simulink model "Controller_damping_cbf_22Franka"  (R2022b)
settings: Solver=FixedStepDiscrete  StartTime=0.0  StopTime=inf  FixedStep=0.001  RelTol=1e-3
PreLoadFcn:
  | set_param(gcs, 'RTWSystemTargetFile', 'franka_emika_panda.tlc');
  | 
  | demos_common_configs();
  | collision_behavior = ones(1,52)*100;
values from neighbouring files (symbols this model uses):
  b_sg = fliplr(B(end, :))    [init_damping_cbf.m]
  cbf_damping_params = [cbf_p_ths; cbf_v_ths; cbf_v_0; cbf_gamma; cbf_d_max;                        cbf_w_lin; cbf_w_quad; plane_normal; plane_offset;                        cbf_latch_entry; cbf_zone_hyst; cbf_latch_alpha; cbf_clip_drift;                        cbf_tau_rate; cbf_dt; cbf_gamma_pos_scale]    [init_damping_cbf.m]
  cbf_kappa = 0.85 * cbf_d_max / cbf_rho_eff    (= 82.6388888889)    [init_damping_cbf.m]
  cbf_stiff_decouple = 0    [init_damping_cbf.m]
  Dn = 20 * ones(7,1)    [init_damping_cbf.m]
  H_home = getTransform(Franka_robot, q_home, 'panda_link8', 'panda_link0')    [init_damping_cbf.m]
  Kn = 0 * ones(7,1)    [init_damping_cbf.m]
  plane_normal = [0.0; 0.0; 1.0]    [init_damping_cbf.m]
  q_home = q_init    [init_damping_cbf.m]
  q_init = [0 0  0  -(2/4)*pi  0  pi/2  -pi/4]'    [init_damping_cbf.m]
undefined symbols (not defined in the file or in its folder): DiscIntNeverNeededParam, Fext_mag
libraries: matrix_library x3, franka_simulink_library x2, Robotics_lib x1
(part 3 of 8)

== matlab function Controller_damping_cbf_22Franka/task space controller/MATLAB Function2 ==
  data: H_IT input; x_c output size=1; v_c output size=1; V_tilde input; lambda_mat input; n_hp input; m_c output size=1; xTableHight input; eef_height input
function [x_c, v_c, m_c] = fcn(H_IT, V_tilde, lambda_mat, n_hp, xTableHight, eef_height)

auxMat = zeros(4,4);
auxMat(3,4) = -xTableHight;

H = H_IT*[eye(3), [0;0;eef_height];zeros(1,3),1] + auxMat;

x_c = transpose(n_hp)*[H(1:3,4);zeros(3,1)];

v_c = transpose(n_hp)*V_tilde;




lambda_inv = lambda_mat\eye(6);
lambda_inv = (lambda_inv + transpose(lambda_inv))./2;

tmp3 = transpose(n_hp)*lambda_inv*n_hp;
m_c = tmp3\eye(1);


end

== matlab function Controller_damping_cbf_22Franka/Dynamic Parameters/End Effector ==
  data: q input; H_0e output
function H_0e = H_0e(q)
% Author: TU Wien, ACIN Robotics group
% Optimized and generated from Maple
  H_0e = zeros(4,4);
  t4449 = q(6);
  t4435 = sin(t4449);
  t4442 = cos(t4449);
  t4431 = 0.107e0 * t4435 + 0.88e-1 * t4442;
  t4450 = q(5);
  t4436 = sin(t4450);
  t4452 = q(3);
  t4438 = sin(t4452);
  t4491 = t4438 * t4436;
  t4499 = t4431 * t4491;
  t4430 = 0.107e0 * t4442 - 0.88e-1 * t4435 - 0.384e0;
  t4451 = q(4);
  t4437 = sin(t4451);
  t4498 = -t4430 * t4437 - 0.825e-1;
  t4443 = cos(t4450);
  t4427 = t4431 * t4443 - 0.825e-1;
  t4444 = cos(t4451);
  t4497 = t4427 * t4444;
  t4495 = t4430 * t4444;
  t4448 = q(7);
  t4434 = sin(t4448);
  t4454 = q(1);
  t4440 = sin(t4454);
  t4494 = t4434 * t4440;
  t4493 = t4436 * t4437;
  t4492 = t4437 * t4435;
  t4490 = t4438 * t4442;
  t4489 = t4438 * t4443;
  t4441 = cos(t4448);
  t4488 = t4440 * t4441;
  t4487 = t4443 * t4437;
  t4486 = t4443 * t4444;
  t4445 = cos(t4452);
  t4485 = t4443 * t4445;
  t4484 = t4444 * t4435;
  t4483 = t4445 * t4436;
  t4482 = t4445 * t4437;
  t4481 = t4445 * t4444;
  t4453 = q(2);
  t4439 = sin(t4453);
  t4446 = cos(t4453);
  t4467 = t4436 * t4481;
  t4458 = (t4467 + t4489) * t4446;
  t4478 = t4434 * t4493;
  t4480 = t4434 * t4458 + t4439 * t4478;
  t4479 = t4431 * t4483;
  t4477 = t4442 * t4487;
  t4476 = t4436 * t4490;
  t4475 = t4444 * t4491;
  t4474 = t4441 * t4493;
  t4473 = t4437 * t4490;
  t4472 = t4442 * t4486;
  t4471 = t4442 * t4483;
  t4470 = t4440 * t4485;
  t4469 = t4438 * t4486;
  t4468 = t4443 * t4481;
  t4466 = t4427 * t4437 + 0.316e0;
  t4465 = t4497 - t4498;
  t4464 = -0.1e1 * t4497 + t4498;
  t4463 = t4477 + t4484;
  t4462 = t4472 - 0.1e1 * t4492;
  t4461 = -0.1e1 * t4472 + t4492;
  t4460 = -0.1e1 * t4477 - 0.1e1 * t4484;
  t4459 = -0.1e1 * t4467 - 0.1e1 * t4489;
  t4447 = cos(t4454);
  t4457 = (t4475 - 0.1e1 * t4485) * t4447;
  t4456 = t4438 * t4462 + t4471;
  t4455 = -0.1e1 * t4471 + t4461 * t4438;
  t4425 = t4445 * t4461 + t4476;
  t4424 = t4462 * t4445 - 0.1e1 * t4476;
  t4423 = ((-0.1e1 * t4491 + t4468) * t4446 + t4439 * t4487) * t4435 + (t4446 * t4482 - 0.1e1 * t4439 * t4444) * t4442;
  t4422 = t4424 * t4446 + t4439 * t4463;
  t4421 = (t4425 * t4446 + t4439 * t4460) * t4434 + t4441 * t4458 + t4439 * t4474;
  t4420 = (t4465 * t4445 - 0.1e1 * t4499) * t4446 + (-0.1e1 * t4495 + t4466) * t4439;
  H_0e(1,3) = t4423 * t4447 + ((-0.1e1 * t4483 - 0.1e1 * t4469) * t4435 - 0.1e1 * t4473) * t4440;
  H_0e(4,1) = 0.0e0;
  H_0e(4,3) = 0.0e0;
  H_0e(3,1) = (t4425 * t4439 + t4446 * t4463) * t4441 + t4459 * t4434 * t4439 + t4446 * t4478;
  H_0e(2,1) = (t4422 * t4440 + t4447 * t4456) * t4441 + t4480 * t4440 + t4434 * t4457;
  H_0e(4,4) = 0.1e1;
  H_0e(3,2) = (t4424 * t4434 + t4441 * t4459) * t4439 + (t4434 * t4460 + t4474) * t4446;
  H_0e(3,4) = (t4445 * t4464 + t4499) * t4439 + 0.333e0 + (t4466 - t4495) * t4446;
  H_0e(2,3) = t4423 * t4440 + ((t4469 + t4483) * t4435 + t4473) * t4447;
  H_0e(2,4) = t4420 * t4440 + (t4438 * t4465 + t4479) * t4447;
  H_0e(4,2) = 0.0e0;
  H_0e(2,2) = t4434 * t4447 * t4455 + t4421 * t4440 + t4441 * t4457;
  H_0e(1,1) = (t4422 * t4441 + t4480) * t4447 + t4455 * t4488 - 0.1e1 * t4475 * t4494 + t4434 * t4470;
  H_0e(3,3) = ((t4491 - 0.1e1 * t4468) * t4435 - 0.1e1 * t4442 * t4482) * t4439 + (-0.1e1 * t4442 * t4444 + t4435 * t4487) * t4446;
  H_0e(1,4) = t4420 * t4447 + (-0.1e1 * t4479 + t4464 * t4438) * t4440;
  H_0e(1,2) = t4421 * t4447 + t4456 * t4494 - 0.1e1 * t4475 * t4488 + t4441 * t4470;
end

== matlab function Controller_damping_cbf_22Franka/Dynamic Parameters/End Effector1 ==
  data: q_state input; H_0e output
function H_0e = Franka_EndEffectorPos(q_state)
% Author: TU Wien, ACIN Robotics group
% Optimized and generated from Maple
  H_0e = zeros(4,4);

  t30 = q_state(6);
  t16 = sin(t30);
  t23 = cos(t30);
  t12 = 0.1070e0 * t16 + 0.88e-1 * t23;
  t31 = q_state(5);
  t17 = sin(t31);
  t33 = q_state(3);
  t19 = sin(t33);
  t71 = t19 * t17;
  t80 = t12 * t71;
  t11 = 0.1070e0 * t23 - 0.88e-1 * t16 - 0.384e0;
  t32 = q_state(4);
  t18 = sin(t32);
  t79 = -t11 * t18 - 0.825e-1;
  t25 = cos(t32);
  t24 = cos(t31);
  t8 = t12 * t24 - 0.825e-1;
  t78 = t8 * t25;
  t29 = q_state(7);
  t15 = sin(t29);
  t34 = q_state(2);
  t20 = sin(t34);
  t27 = cos(t34);
  t26 = cos(t33);
  t61 = t26 * t25;
  t57 = t17 * t61;
  t69 = t19 * t24;
  t39 = (t57 + t69) * t27;
  t72 = t17 * t18;
  t60 = t15 * t72;
  t77 = t15 * t39 + t20 * t60;
  t75 = t11 * t25;
  t35 = q_state(1);
  t21 = sin(t35);
  t74 = t15 * t21;
  t73 = t18 * t16;
  t70 = t19 * t23;
  t22 = cos(t29);
  t68 = t21 * t22;
  t67 = t24 * t18;
  t66 = t24 * t26;
  t65 = t16 * t25;
  t64 = t25 * t24;
  t63 = t26 * t17;
  t62 = t26 * t18;
  t59 = t12 * t63;
  t58 = t25 * t71;
  t56 = t17 * t70;
  t55 = t22 * t72;
  t54 = t18 * t70;
  t53 = t23 * t67;
  t52 = t23 * t64;
  t51 = t23 * t63;
  t50 = t21 * t66;
  t49 = t19 * t64;
  t48 = t24 * t61;
  t47 = t8 * t18 + 0.316e0;
  t46 = t78 - t79;
  t45 = t53 + t65;
  t44 = -0.1e1 * t73 + t52;
  t43 = -0.1e1 * t52 + t73;
  t42 = -0.1e1 * t78 + t79;
  t41 = -0.1e1 * t57 - 0.1e1 * t69;
  t40 = -0.1e1 * t53 - 0.1e1 * t65;
  t28 = cos(t35);
  t38 = (t58 - 0.1e1 * t66) * t28;
  t37 = t19 * t44 + t51;
  t36 = -0.1e1 * t51 + t43 * t19;
  t6 = t26 * t43 + t56;
  t5 = t44 * t26 - 0.1e1 * t56;
  t4 = ((-0.1e1 * t71 + t48) * t27 + t20 * t67) * t16 + (t27 * t62 - 0.1e1 * t20 * t25) * t23;
  t3 = t20 * t45 + t27 * t5;
  t2 = (t20 * t40 + t27 * t6) * t15 + t22 * t39 + t20 * t55;
  t1 = (t46 * t26 - 0.1e1 * t80) * t27 + (-0.1e1 * t75 + t47) * t20;
  H_0e(2,3) = t4 * t21 + ((t49 + t63) * t16 + t54) * t28;
  H_0e(3,3) = ((t71 - 0.1e1 * t48) * t16 - 0.1e1 * t23 * t62) * t20 + (t16 * t67 - 0.1e1 * t23 * t25) * t27;
%   H_0e(4,2) = 0.0e0;
  H_0e(2,4) = t1 * t21 + (t19 * t46 + t59) * t28;
%   H_0e(4,1) = 0.0e0;
  H_0e(2,2) = t15 * t28 * t36 + t2 * t21 + t22 * t38;
  H_0e(1,3) = t4 * t28 + ((-0.1e1 * t63 - 0.1e1 * t49) * t16 - 0.1e1 * t54) * t21;
  H_0e(1,2) = t2 * t28 + t37 * t74 - 0.1e1 * t58 * t68 + t22 * t50;
  H_0e(3,2) = (t15 * t5 + t22 * t41) * t20 + (t15 * t40 + t55) * t27;
  H_0e(1,4) = t1 * t28 + (-0.1e1 * t59 + t42 * t19) * t21;
  H_0e(1,1) = (t22 * t3 + t77) * t28 + t36 * t68 - 0.1e1 * t58 * t74 + t15 * t50;
  H_0e(2,1) = (t21 * t3 + t28 * t37) * t22 + t77 * t21 + t15 * t38;
  H_0e(4,4) = 1;
  H_0e(3,1) = (t20 * t6 + t27 * t45) * t22 + t41 * t15 * t20 + t27 * t60;
%   H_0e(4,3) = 0.0e0;
  H_0e(3,4) = (t26 * t42 + t80) * t20 + 0.333e0 + (t47 - t75) * t27;
end

== matlab function Controller_damping_cbf_22Franka/Dynamic Parameters/Geometric Jacobian ==
  data: q input; J_geo output
function J_geo = J_geometric(q)
% Author: TU Wien, ACIN Robotics group
% Optimized and generated from Maple
  J_geo = zeros(6,7);
  t4550 = q(3);
  t4544 = cos(t4550);
  t4549 = q(4);
  t4537 = sin(t4549);
  t4547 = q(6);
  t4535 = sin(t4547);
  t4532 = 0.88e-1 * t4535 + 0.384e0;
  t4541 = cos(t4547);
  t4571 = 0.107e0 * t4541;
  t4616 = -t4532 + t4571;
  t4621 = t4616 * t4537;
  t4513 = -0.825e-1 - t4621;
  t4543 = cos(t4549);
  t4584 = 0.88e-1 * t4541;
  t4527 = 0.107e0 * t4535 + t4584;
  t4548 = q(5);
  t4542 = cos(t4548);
  t4558 = t4527 * t4542 - 0.825e-1;
  t4610 = t4558 * t4543;
  t4623 = -t4610 + t4513;
  t4504 = t4623 * t4544;
  t4536 = sin(t4548);
  t4538 = sin(t4550);
  t4604 = t4538 * t4536;
  t4625 = t4527 * t4604 + t4504;
  t4567 = 0.10700e0 * t4535;
  t4514 = 0.82500e-1 + (-t4567 - t4584) * t4542;
  t4585 = 0.88e-1 * t4538;
  t4565 = t4536 * t4585;
  t4530 = t4541 * t4565;
  t4551 = q(2);
  t4539 = sin(t4551);
  t4545 = cos(t4551);
  t4560 = t4536 * t4567;
  t4615 = t4532 - 0.10700e0 * t4541;
  t4619 = ((t4514 * t4543 + t4537 * t4615 - 0.82500e-1) * t4544 + t4538 * t4560 + t4530) * t4539 + (-t4514 * t4537 + t4543 * t4615 + 0.316e0) * t4545;
  t4611 = t4558 * t4537;
  t4591 = t4545 * t4544;
  t4508 = (t4537 * t4539 + t4543 * t4591) * t4536 + t4545 * t4538 * t4542;
  t4552 = q(1);
  t4540 = sin(t4552);
  t4546 = cos(t4552);
  t4590 = t4546 * t4538;
  t4617 = t4536 * t4543 * t4590 + t4508 * t4540;
  t4606 = t4616 * t4543;
  t4554 = -t4606 + t4611;
  t4531 = 0.13375e2 * t4535 + 0.11e2 * t4541;
  t4613 = -0.8e-2 * t4531;
  t4570 = 0.107e0 * t4543;
  t4561 = t4542 * t4570;
  t4586 = 0.88e-1 * t4537;
  t4609 = (t4561 - t4586) * t4544;
  t4583 = 0.88e-1 * t4543;
  t4564 = t4542 * t4583;
  t4573 = 0.107e0 * t4537;
  t4608 = (t4564 + t4573) * t4544;
  t4605 = t4535 * t4537;
  t4603 = t4544 * t4539;
  t4602 = t4538 * t4540;
  t4601 = t4539 * t4540;
  t4600 = t4540 * t4543;
  t4599 = t4540 * t4544;
  t4598 = t4540 * t4545;
  t4597 = t4541 * t4537;
  t4596 = t4542 * t4539;
  t4595 = t4542 * t4543;
  t4594 = t4544 * t4536;
  t4593 = t4544 * t4543;
  t4592 = t4545 * t4537;
  t4589 = t4546 * t4539;
  t4588 = t4546 * t4544;
  t4519 = t4527 * t4594;
  t4582 = t4538 * t4600;
  t4581 = t4538 * t4596;
  t4580 = t4539 * t4593;
  t4579 = t4538 * t4597;
  t4578 = t4538 * t4595;
  t4577 = t4542 * t4593;
  t4576 = t4542 * t4588;
  t4575 = t4545 * t4590;
  t4574 = t4545 * t4588;
  t4572 = 0.107e0 * t4538;
  t4563 = 0.88e-1 * t4594;
  t4562 = t4536 * t4572;
  t4559 = -0.316e0 + t4606;
  t4556 = (-t4537 * t4585 + t4538 * t4561 + 0.107e0 * t4594) * t4541 - (t4537 * t4572 + t4538 * t4564 + t4563) * t4535;
  t4553 = (t4542 * t4573 + t4583) * t4541 + (-t4542 * t4586 + t4570) * t4535;
  t4533 = t4542 * t4599;
  t4503 = ((-0.1e1 * t4604 + t4577) * t4545 + t4537 * t4596) * t4535 + (t4537 * t4591 - 0.1e1 * t4539 * t4543) * t4541;
  t4502 = t4538 * t4623 - t4519;
  t4501 = -t4554 * t4591 + (t4610 + (t4571 - 0.1e1 * t4532) * t4537) * t4539;
  t4500 = ((-t4562 + t4609) * t4541 + (t4565 - 0.1e1 * t4608) * t4535) * t4545 + t4553 * t4539;
  J_geo(1,3) = t4502 * t4545 * t4546 + t4540 * t4625;
  J_geo(3,5) = 0.8e-2 * (t4581 + (t4580 - t4592) * t4536) * t4531;
  J_geo(6,4) = -0.1e1 * t4539 * t4538;
  J_geo(3,7) = 0.0e0;
  J_geo(4,1) = 0.0e0;
  J_geo(4,3) = t4589;
  J_geo(5,1) = 0.0e0;
  J_geo(5,6) = -0.1e1 * t4576 + t4617;
  J_geo(2,6) = t4500 * t4540 + t4546 * t4556;
  J_geo(4,5) = (-0.1e1 * t4574 + t4602) * t4537 + t4543 * t4589;
  J_geo(5,4) = t4538 * t4598 - 0.1e1 * t4588;
  J_geo(3,1) = 0.0e0;
  J_geo(6,3) = t4545;
  J_geo(4,7) = t4503 * t4546 + ((-0.1e1 * t4594 - 0.1e1 * t4578) * t4535 - 0.1e1 * t4579) * t4540;
  J_geo(6,7) = ((t4604 - 0.1e1 * t4577) * t4535 - 0.1e1 * t4544 * t4597) * t4539 + (-0.1e1 * t4543 * t4541 + t4542 * t4605) * t4545;
  J_geo(3,6) = ((t4562 - 0.1e1 * t4609) * t4541 + (-t4565 + t4608) * t4535) * t4539 + t4553 * t4545;
  J_geo(5,2) = t4546;
  J_geo(2,1) = (-t4625 * t4545 + (-0.1e1 * t4606 + t4611 + 0.316e0) * t4539) * t4546 - t4540 * t4519 - t4558 * t4582 + t4513 * t4602;
  J_geo(4,4) = t4575 + t4599;
  J_geo(5,5) = (-0.1e1 * t4540 * t4591 - 0.1e1 * t4590) * t4537 + t4539 * t4600;
  J_geo(6,5) = t4537 * t4603 + t4543 * t4545;
  J_geo(3,2) = (t4535 * t4562 + t4504 + t4530) * t4545 + (t4559 - t4611) * t4539;
  J_geo(3,4) = (t4621 + t4610) * t4545 + t4554 * t4603;
  J_geo(4,6) = t4508 * t4546 + t4533 - 0.1e1 * t4536 * t4582;
  J_geo(2,3) = t4502 * t4598 - t4546 * t4625;
  J_geo(2,7) = 0.0e0;
  J_geo(2,5) = (-t4576 + t4617) * t4613;
  J_geo(1,7) = 0.0e0;
  J_geo(2,4) = t4501 * t4540 - t4554 * t4590;
  J_geo(4,2) = -0.1e1 * t4540;
  J_geo(2,2) = t4540 * t4619;
  J_geo(1,1) = t4625 * t4598 + (-0.1e1 * t4519 + (-0.1e1 * t4610 + t4513) * t4538) * t4546 + (-0.1e1 * t4611 + t4559) * t4601;
  J_geo(5,3) = t4601;
  J_geo(6,1) = 0.1e1;
  J_geo(3,3) = (t4544 * t4560 - 0.1e1 * (-0.1e1 * t4541 * t4595 + t4605) * t4585 + t4563 * t4541 + (-0.384e0 * t4537 - 0.82500e-1 * t4543 + 0.82500e-1 + 0.10700e0 * t4535 * t4595 + 0.10700e0 * t4597) * t4538) * t4539;
  J_geo(5,7) = t4503 * t4540 + ((t4578 + t4594) * t4535 + t4579) * t4546;
  J_geo(1,5) = (t4542 * t4575 + t4533 + (t4537 * t4589 + (t4574 - t4602) * t4543) * t4536) * t4613;
  J_geo(6,2) = 0.0e0;
  J_geo(1,4) = t4501 * t4546 + t4554 * t4602;
  J_geo(1,2) = t4546 * t4619;
  J_geo(1,6) = t4500 * t4546 - t4540 * t4556;
  J_geo(6,6) = (-0.1e1 * t4580 + t4592) * t4536 - 0.1e1 * t4581;
end

== matlab function Controller_damping_cbf_22Franka/MATLAB Function4 ==
  data: H_IT input; p_data output; q_dot input; p_dot_data output; Jg_mat input
function [p_data, p_dot_data] = fcn(H_IT, q_dot, Jg_mat)

p_data = H_IT(1:3,4);

V = Jg_mat*q_dot;
p_dot_data = V(1:3);

end

== matlab function Controller_damping_cbf_22Franka/Dynamic Parameters/Geometric Jacobian Derivative ==
  data: q input; J_geo_dot output; q_dot input
function J_geo_dot = J_geometric_dot(q, q_dot)
% Author: TU Wien, ACIN Robotics group
% Optimized and generated from Maple
  J_geo_dot = zeros(6,7);
  t4800 = q_dot(4);
  t4783 = 0.825e-1 * t4800;
  t4806 = q(4);
  t4788 = sin(t4806);
  t4804 = q(6);
  t4792 = cos(t4804);
  t4805 = q(5);
  t4787 = sin(t4805);
  t4799 = q_dot(5);
  t4932 = 0.88e-1 * t4799;
  t4767 = t4787 * t4932;
  t4903 = 0.107e0 * t4800;
  t4726 = -t4767 + t4903;
  t4793 = cos(t4805);
  t4798 = q_dot(6);
  t4905 = 0.107e0 * t4798;
  t4860 = t4793 * t4905;
  t5026 = t4726 + t4860;
  t4782 = 0.384e0 * t4800;
  t4786 = sin(t4804);
  t4904 = 0.107e0 * t4799;
  t4931 = 0.88e-1 * t4800;
  t4725 = t4787 * t4904 + t4931;
  t4933 = 0.88e-1 * t4798;
  t4765 = t4793 * t4933;
  t4835 = t4725 + t4765;
  t5041 = t4786 * t4835 + t4782;
  t4643 = -t4792 * t5026 + t5041;
  t4794 = cos(t4806);
  t4638 = t4643 * t4794;
  t4872 = t4793 * t4931;
  t4727 = t4872 + t4933;
  t4801 = q_dot(3);
  t4930 = 0.88e-1 * t4801;
  t4769 = t4787 * t4930;
  t4662 = (t4727 * t4788 + t4769) * t4792;
  t4947 = -t4638 - t4662;
  t5048 = -t4783 * t4788 - t4947;
  t4808 = q(2);
  t4790 = sin(t4808);
  t4803 = q_dot(1);
  t4928 = 0.88e-1 * t4803;
  t4773 = t4790 * t4928;
  t4807 = q(3);
  t4789 = sin(t4807);
  t5035 = t4835 * t4789;
  t4655 = t4773 - t5035;
  t5047 = t4655 * t4786;
  t4970 = t4793 * t4800;
  t5046 = t4798 + t4970;
  t4776 = t4799 * t4789;
  t4802 = q_dot(2);
  t4779 = t4802 * t4788;
  t4966 = t4794 * t4801;
  t4919 = t4789 * t4966;
  t4795 = cos(t4807);
  t4963 = t4795 * t4800;
  t4921 = t4788 * t4963;
  t4661 = -0.1e1 * t4919 - 0.1e1 * t4921 + t4779 - 0.1e1 * t4776;
  t4957 = t4802 * t4789;
  t4960 = t4799 * t4788;
  t4735 = -0.1e1 * t4957 + t4960;
  t4777 = t4799 * t4794;
  t4745 = t4777 + t4801;
  t4796 = cos(t4808);
  t4950 = t4803 * t4795;
  t4965 = t4795 * t4796;
  t4981 = t4790 * t4793;
  t4736 = -0.1e1 * t4803 * t4789 + t4790 * t4800;
  t4780 = t4802 * t4795;
  t4917 = t4790 * t4780;
  t5021 = -0.1e1 * t4917 + t4736;
  t4632 = t4735 * t4981 + (t4661 * t4796 + t4794 * t5021) * t4787 + (t4745 * t4965 + t4950) * t4793;
  t4952 = t4803 * t4790;
  t4748 = t4788 * t4952;
  t4959 = t4800 * t4789;
  t4924 = t4788 * t4959;
  t4700 = -0.1e1 * t4748 + t4924;
  t4809 = q(1);
  t4791 = sin(t4809);
  t4797 = cos(t4809);
  t4978 = t4791 * t4795;
  t4825 = (-0.1e1 * t4799 - 0.1e1 * t4966) * t4978;
  t4781 = t4803 * t4796;
  t4852 = -0.1e1 * t4781 - 0.1e1 * t4801;
  t4916 = t4791 * t4781;
  t4969 = t4794 * t4795;
  t4974 = t4793 * t4791;
  t5045 = (-0.1e1 * t4916 * t4969 + t4825 + t4700 * t4791) * t4787 + (-0.1e1 * t4777 + t4852) * t4789 * t4974 + t4632 * t4797;
  t4896 = 0.107e0 * t4803;
  t4763 = t4790 * t4896;
  t5036 = t4789 * t5026;
  t4654 = t4763 - t5036;
  t4753 = t4789 * t4782;
  t4894 = 0.384e0 * t4803;
  t4854 = t4790 * t4894;
  t5044 = t4654 * t4792 + t4753 - t4854;
  t5025 = t4781 + t4801;
  t4844 = t5025 * t4794;
  t4850 = -0.1e1 * t4924 + t4748;
  t4983 = t4789 * t4797;
  t5043 = ((t4799 + t4844) * t4795 + t4850) * t4797 * t4787 + (t4777 + t5025) * t4793 * t4983 + t4632 * t4791;
  t4901 = 0.107e0 * t4801;
  t4855 = t4789 * t4901;
  t4929 = 0.88e-1 * t4802;
  t4712 = -t4793 * t4855 + t4929;
  t4874 = t4789 * t4930;
  t4899 = 0.107e0 * t4802;
  t4713 = t4793 * t4874 + t4899;
  t4902 = 0.825e-1 * t4801;
  t4758 = t4789 * t4902;
  t4784 = 0.384e0 * t4802;
  t4867 = t4712 * t4786 - t4713 * t4792 + t4758 + t4784;
  t5042 = t4643 * t4795 - t4867;
  t5040 = t4867 * t4794 + 0.316e0 * t4802;
  t4934 = 0.88e-1 * t4793;
  t4742 = t4792 * t4934;
  t4892 = 0.10700e0 * t4786;
  t4813 = t4793 * t4892 + t4742 - 0.82500e-1;
  t5032 = -t4813 * t4788 - 0.316e0;
  t5031 = t4813 * t4794 + 0.82500e-1;
  t4766 = t4787 * t4933;
  t4717 = t4793 * t4904 - t4766;
  t4770 = t4788 * t4930;
  t5034 = -(t4717 - t4770) * t4786 - t4902;
  t4858 = t4793 * t4903;
  t5033 = t4788 * t4858 + t4794 * t4835;
  t4774 = 0.88e-1 * t4786;
  t4834 = 0.384e0 + t4774;
  t4891 = 0.10700e0 * t4792;
  t4722 = t4891 - t4834;
  t4647 = -t4722 * t4788 - t5031;
  t5029 = t4647 * t4795;
  t5001 = t4717 * t4786;
  t4935 = 0.88e-1 * t4792;
  t4824 = 0.107e0 * t4786 + t4935;
  t5028 = t4794 * (-t4824 * t4793 + 0.825e-1);
  t4817 = t4824 * t4802;
  t5027 = t4834 * t4788;
  t4724 = t4858 + t4905;
  t4997 = t4724 * t4786;
  t4943 = -t4997 + t4783;
  t4912 = -t4727 * t4792 + t4943;
  t4658 = t4803 * t5028;
  t4754 = t4787 * t4901;
  t4738 = t4786 * t4754;
  t4908 = 0.107e0 * t4792;
  t4823 = -t4908 + t4774;
  t4897 = 0.825e-1 * t4803;
  t4764 = t4790 * t4897;
  t4856 = t4789 * t4783;
  t4831 = t4764 - t4856;
  t4865 = t4787 * t4896;
  t4840 = t4786 * t4865;
  t4990 = t4787 * t4789;
  t4876 = 0.88e-1 * t4990;
  t4843 = t4792 * t4876;
  t4988 = t4788 * t4789;
  t5024 = ((t4658 + (-0.825e-1 + (t4823 + 0.384e0) * t4788) * t4803) * t4795 + t4789 * t4840 + t4803 * t4843) * t4796 + (t5044 - t5047) * t4794 + ((t4724 * t4789 - t4763 * t4793) * t4786 + t4831) * t4788 + (-t4773 * t4788 * t4793 + t4727 * t4988 + t4769 * t4789) * t4792 + t4789 * t4738;
  t4900 = 0.384e0 * t4801;
  t4755 = t4788 * t4900;
  t4657 = t4801 * t5028;
  t4751 = t4787 * t4905;
  t4710 = t4788 * t4901 + t4751;
  t4768 = t4793 * t4932;
  t4665 = (t4710 + t4768) * t4792;
  t4944 = t4657 - t4665;
  t5023 = t4755 + t4944 + t5034;
  t5022 = t4780 - 0.1e1 * t4800;
  t4785 = 0.825e-1 * t4802;
  t4759 = t4790 * t4785;
  t4652 = (-t4817 * t4981 + t4759) * t4794;
  t4761 = t4789 * t4896;
  t4847 = t5046 * t4790;
  t5020 = (-t4793 * t4761 + 0.107e0 * t4847) * t4786;
  t4772 = t4789 * t4928;
  t4994 = t4772 * t4793;
  t5019 = (0.88e-1 * t4847 - t4994) * t4792;
  t4890 = 0.10700e0 * t4798;
  t5018 = (t4793 * t4890 - t4767 + 0.10700e0 * t4800) * t4792;
  t4953 = t4803 * t4787;
  t5017 = t4824 * t4953 * t4796;
  t5016 = t5026 * t4794;
  t4694 = 0.10700000000000000000e0 * t5046;
  t5013 = t4694 * t4786;
  t4695 = 0.88000000000000000000e-1 * t5046;
  t5012 = t4695 * t4792;
  t4956 = t4802 * t4790;
  t5011 = t4956 * t5027;
  t4861 = t4790 * t4899;
  t4878 = t4787 * t4928;
  t4675 = (t4788 * t4861 + t4878) * t4792;
  t5010 = (t4788 * t4899 - t4789 * t4904) * t4793;
  t5009 = (-t4789 * t4903 + t4763) * t4793;
  t5007 = t4712 * t4794;
  t5005 = t4713 * t4794;
  t5004 = (t4793 * t4899 + t4874) * t4786;
  t4871 = t4793 * t4929;
  t4715 = -t4855 + t4871;
  t5003 = t4715 * t4788;
  t4692 = t4715 * t4792;
  t4716 = -t4751 - t4768;
  t5002 = t4716 * t4789;
  t4771 = t4788 * t4929;
  t5000 = (t4789 * t4932 - t4771) * t4793;
  t4999 = (t4789 * t4931 - t4773) * t4793;
  t4998 = t4722 * t4794;
  t4996 = t4724 * t4788;
  t4995 = (0.13375e2 * t4792 - 0.11e2 * t4786) * t4798;
  t4993 = t4786 * t4795;
  t4992 = t4786 * t4796;
  t4991 = t4786 * t4797;
  t4989 = t4787 * t4790;
  t4987 = t4788 * t4792;
  t4986 = t4788 * t4796;
  t4985 = t4789 * t4791;
  t4984 = t4789 * t4792;
  t4982 = t4790 * t4788;
  t4980 = t4790 * t4801;
  t4979 = t4791 * t4794;
  t4976 = t4792 * t4796;
  t4975 = t4792 * t4797;
  t4973 = t4793 * t4794;
  t4972 = t4793 * t4795;
  t4971 = t4793 * t4798;
  t4968 = t4794 * t4796;
  t4967 = t4794 * t4797;
  t4964 = t4795 * t4797;
  t4962 = t4796 * t4797;
  t4961 = t4798 * t4787;
  t4775 = t4798 * t4788;
  t4958 = t4801 * t4788;
  t4955 = t4802 * t4794;
  t4954 = t4802 * t4796;
  t4951 = t4803 * t4791;
  t4949 = t4803 * t4797;
  t4946 = t4638 + t4738;
  t4760 = t4789 * t4894;
  t4945 = (-t4790 * t4835 + t4772) * t4786 + t4760;
  t4942 = t4787 * t4890 + t4768;
  t4752 = t4788 * t4905;
  t4708 = -t4752 - t4754;
  t4718 = t4766 + t4770;
  t4778 = t4801 * t4787;
  t4940 = t4778 + t4775;
  t4939 = t4785 - t5004;
  t4889 = 0.10700e0 * t4799;
  t4938 = t4793 * t4889 - 0.1e1 * t4766;
  t4937 = -0.1e1 * t4778 - 0.1e1 * t4775;
  t4936 = 0.88e-1 * t4788;
  t4927 = t4789 * t5001;
  t4925 = t4789 * t4971;
  t4923 = t4793 * t4969;
  t4920 = t4787 * t4777;
  t4918 = t4789 * t4956;
  t4915 = -0.8e-2 * t4995;
  t4913 = t4675 + t4759 - t4652;
  t4910 = 0.107e0 * t4787;
  t4909 = 0.107e0 * t4788;
  t4907 = 0.107e0 * t4793;
  t4906 = 0.107e0 * t4795;
  t4895 = 0.316e0 * t4803;
  t4888 = 0.82500e-1 * t4800;
  t4887 = 0.10700e0 * t4801;
  t4756 = t4789 * t4900;
  t4886 = t5004 + t4756 - 0.1e1 * t4785;
  t4885 = -0.1e1 * t4756 + t4939;
  t4884 = (t4787 * t4889 + t4765 + t4931) * t4786 + t4782;
  t4882 = t4799 + t4966;
  t4880 = t4796 * t4801 + t4803;
  t4879 = -0.1e1 * t4780 + t4800;
  t4877 = t4788 * t4928;
  t4875 = t4789 * t4933;
  t4873 = t4794 * t4934;
  t4870 = t4789 * t4920;
  t4864 = t4788 * t4896;
  t4863 = t4789 * t4910;
  t4862 = t4789 * t4905;
  t4853 = -0.1e1 * t4970 - 0.1e1 * t4798;
  t4851 = t4787 * t4892;
  t4848 = t4795 * t4880;
  t4846 = t4882 * t4793;
  t4845 = t5025 * t4788;
  t4842 = t4802 * t4876;
  t4841 = -t4952 + t4959;
  t4838 = 0.10700000000000000000e0 * t4786 + 0.88000000000000000000e-1 * t4792;
  t4837 = t4957 - 0.1e1 * t4960;
  t4721 = t4788 * t4933 + t4769;
  t4830 = t4758 - t5040;
  t4749 = t4788 * t4894;
  t4829 = t4658 + t4749 - t4897;
  t4828 = t4788 * t4852;
  t4826 = -0.1e1 * t4923 + t4990;
  t4821 = t4891 - t4774;
  t4820 = (-t4860 - 0.1e1 * t4726) * t4788;
  t4819 = -0.1e1 * t4773 + t5035;
  t4818 = -0.1e1 * t4763 + t5036;
  t4816 = t4787 * (t4892 + t4935);
  t4815 = t4919 + t4921 - 0.1e1 * t4779 + t4776;
  t4811 = t4788 * t4906 + t4795 * t4873 - t4876;
  t4810 = -t4795 * t4936 + t4906 * t4973 - t4863;
  t4762 = t4789 * t4897;
  t4750 = t4790 * t4783;
  t4739 = t4792 * t4769;
  t4734 = t4959 - 0.1e1 * t4952;
  t4733 = -0.1e1 * t4959 + t4952;
  t4731 = -0.1e1 * t4961 - 0.1e1 * t4958;
  t4723 = -t4834 + t4908;
  t4707 = t4790 * t4903 - t4761;
  t4698 = t4787 * t4861 + t4877;
  t4697 = t4929 * t4989 - t4864;
  t4686 = t4786 * t4907 + t4742 - 0.825e-1;
  t4682 = t4841 * t4936;
  t4680 = t4802 * t4823 + t4784;
  t4677 = t4841 * t4909;
  t4668 = t4793 * t4817 - t4785;
  t4664 = 0.88e-1 * t4790 * t4853 + t4994;
  t4653 = t4790 * t5026 - t4761;
  t4646 = (t4789 * t4880 + t4790 * t5022) * t4788 + (-0.1e1 * t4963 + t4802) * t4968;
  t4645 = -t4888 + t5012 + t5013;
  t4640 = -t4884 + t5018;
  t4633 = -0.1e1 * t5001 + (-0.825e-1 + t5027) * t4801 + t4944;
  t4631 = (t4754 + t4996) * t4786 + t5048;
  t4630 = (((-0.1e1 * t4920 + t4937) * t4795 + t4661 * t4793) * t4796 + (-0.1e1 * t4953 - 0.1e1 * t4955 * t4981) * t4795 + (t4736 * t4793 + t4790 * t4798) * t4794 + t4787 * t4918 - 0.1e1 * t4960 * t4989) * t4786 + (t4731 * t4789 + ((t4800 + t4971) * t4795 - 0.1e1 * t4802) * t4794) * t4976 + t4792 * t4775 * t4981 + t5021 * t4987;
  t4629 = (t4631 * t4796 + (-t4771 * t4790 + t4865) * t4786 - t4784 * t4982 + t4913) * t4789 + (t4697 * t4792 + t4698 * t4786 + t4796 * t5023 + t4829) * t4795;
  t4628 = (t5042 * t4796 + t4686 * t4917 + t4664 * t4792 + (-t4707 * t4793 - t4790 * t4905) * t4786 - t4762 + t4750) * t4788 + (((-0.1e1 * t5013 - 0.1e1 * t5012 + t4783) * t4795 + t4692 + t4886) * t4796 + t4653 * t4792 + (-0.1e1 * t4723 * t4780 - t4782) * t4790 + t4945) * t4794;
  t4627 = (((-0.1e1 * t4752 - 0.1e1 * t4754 - t5033) * t4795 + t5007 + t5010 + t4718 * t4789) * t4796 - t4795 * t4865 + t4707 * t4973 + t4698 * t4789) * t4792 + (((t4788 * t4872 - 0.1e1 * t5016 + t4721) * t4795 + t5005 + t5000 + t4710 * t4789) * t4796 + t4795 * t4878 + t4664 * t4794 - 0.1e1 * t4697 * t4789) * t4786 + ((t4871 * t4993 + (-0.1e1 * t4793 * t4780 + t4798) * t4908) * t4794 + (-0.1e1 * t4725 * t4792 - 0.1e1 * t4726 * t4786 + t4824 * (t4780 - 0.1e1 * t4971)) * t4788) * t4790;
  t4626 = (((-0.1e1 * t5018 + t4884) * t4794 + t4645 * t4788 + t4801 * t4851 + t4739) * t4795 - 0.1e1 * t4784 * t4794 - 0.1e1 * t4756 * t4788) * t4790 + (t4640 * t4788 + t4645 * t4794) * t4796 + ((t4794 * t4821 + t5032) * t4790 + t4647 * t4965) * t4802 + ((t4786 * t4938 + t4792 * t4942) * t4790 + t4816 * t4954 + (t4788 * t4821 + t5031) * t4980) * t4789;
  J_geo_dot(1,3) = t4629 * t4797 + ((-0.1e1 * t4658 - 0.1e1 * t4749) * t4796 - 0.1e1 * t4657 + t4665 - 0.1e1 * t4755 + (-t4823 * t4788 + 0.825e-1) * t4781 - t5034) * t4985 + (t4631 + t5017) * t4978;
  J_geo_dot(3,5) = ((t4661 * t4787 + t4745 * t4972) * t4790 + (t4787 * t4794 * t5022 + t4793 * t4837) * t4796) * t4838 + (-t4789 * t4981 + (-t4790 * t4969 + t4986) * t4787) * t4915;
  J_geo_dot(6,4) = -0.1e1 * t4789 * t4954 - 0.1e1 * t4795 * t4980;
  J_geo_dot(3,7) = 0.0e0;
  J_geo_dot(4,1) = 0.0e0;
  J_geo_dot(4,3) = -0.1e1 * t4790 * t4951 + t4797 * t4954;
  J_geo_dot(5,1) = 0.0e0;
  J_geo_dot(5,6) = t5043;
  J_geo_dot(2,6) = t4627 * t4791 + (t4810 * t4781 + (-t4718 + 0.107e0 * t4846) * t4795 + t4655 * t4794 - t4677 * t4793 + t4708 * t4789) * t4975 + (-t4811 * t4781 + ((-t4873 - t4909) * t4801 + t4716) * t4795 + t4654 * t4794 + t4682 * t4793 + t4721 * t4789) * t4991;
  J_geo_dot(4,5) = t4646 * t4797 + (t4734 * t4794 + t4795 * t4845) * t4791;
  J_geo_dot(5,4) = (-0.1e1 * t4918 + t4848) * t4791 + t5025 * t4983;
  J_geo_dot(3,1) = 0.0e0;
  J_geo_dot(6,3) = -t4956;
  J_geo_dot(4,7) = t4630 * t4797 + (t4700 * t4974 + t4791 * t4870 + t4793 * t4825 + t4826 * t4916 + t4940 * t4985) * t4786 + ((-0.1e1 * t4925 + t4733) * t4979 + (-0.1e1 * t4788 * t4916 + t4731 * t4791) * t4795) * t4792;
  J_geo_dot(6,7) = (((t4920 + t4940) * t4795 + t4815 * t4793) * t4786 + (t4958 + t4961) * t4984 + ((-0.1e1 * t4971 - 0.1e1 * t4800) * t4969 + t4955) * t4792) * t4790 + ((t4793 * t4879 + t4798) * t4794 + t4837 * t4787) * t4992 + (t4879 + t4971) * t4788 * t4976;
  J_geo_dot(3,6) = (((-t4708 + t5033) * t4795 - 0.1e1 * t5007 - 0.1e1 * t5010) * t4792 + ((t5016 - 0.1e1 * t4769) * t4795 - 0.1e1 * t5005 - 0.1e1 * t5000 - t4788 * t4855 - t4789 * t4751) * t4786 - t4798 * t4843 + (-0.1e1 * t4801 * t4984 + t4853 * t4993) * t4936) * t4790 + (t4724 * t4794 + t4771 * t4795 + t4826 * t4899 + (-t4765 - 0.1e1 * t4725) * t4788) * t4976 + (-0.1e1 * t4727 * t4794 + t4820 + t4811 * t4802) * t4992;
  J_geo_dot(5,2) = -0.1e1 * t4951;
  J_geo_dot(2,1) = (((t4943 * t4788 - 0.1e1 * t4738 + t4947) * t4795 + (t5002 + t5003) * t4792 + t4886 * t4788 - 0.1e1 * t4927 - 0.1e1 * t4758 + t5040) * t4796 + (t4652 + t5011 - 0.1e1 * t4675 - 0.1e1 * t4759) * t4795 + (t5020 + t5019 - 0.1e1 * t4750 + t4762) * t4794 + (t4653 * t4788 + t4790 * t4842) * t4792 + (-0.1e1 * t4790 * t4782 + t4945) * t4788 - 0.1e1 * t4762 + (-0.1e1 * t4950 + t4918) * t4786 * t4910) * t4797 + t4633 * t4978 + (-0.1e1 * t4790 * t4895 + t5024) * t4791;
  J_geo_dot(4,4) = (t4848 - t4918) * t4797 - t5025 * t4985;
  J_geo_dot(5,5) = t4646 * t4791 + t4733 * t4967 + t4828 * t4964;
  J_geo_dot(6,5) = (-t4789 * t4958 - t4794 * (t4802 - t4963)) * t4790 + (t4780 - t4800) * t4986;
  J_geo_dot(3,2) = ((-t4788 * t4912 + t4739 + t4946) * t4795 + (-t4692 + t4885) * t4788 + (-t4716 * t4792 + t5001) * t4789 + t4830) * t4796 + ((t4668 * t4794 - t4680 * t4788 + t4785) * t4795 + t4912 * t4794 + t4643 * t4788 - t4817 * t4990) * t4790;
  J_geo_dot(3,4) = ((-t4795 * t4912 - t4692 - t4756 + t4939) * t4794 - t5042 * t4788) * t4790 + ((t4680 * t4795 - t4643) * t4794 + (t4668 * t4795 + t4912) * t4788) * t4796;
  J_geo_dot(4,6) = t5045;
  J_geo_dot(2,3) = t4629 * t4791 + (((t4786 * t4877 - t4792 * t4864 + t4829) * t4796 + t5023) * t4789 + (-0.1e1 * t5017 + (-0.1e1 * t4996 - 0.1e1 * t4754) * t4786 - t5048) * t4795) * t4797;
  J_geo_dot(2,7) = 0.0e0;
  J_geo_dot(2,5) = -t5043 * t4838 + 0.8e-2 * ((-t4796 * t4985 + t4964) * t4793 + (-t4789 * t4967 + (-t4794 * t4965 - t4982) * t4791) * t4787) * t4995;
  J_geo_dot(1,7) = 0.0e0;
  J_geo_dot(2,4) = t4628 * t4791 + ((t4786 * t4819 + t5044) * t4788 + ((-t4875 - 0.1e1 * t4999) * t4792 + (-t4862 + t5009) * t4786 + t4856 - 0.1e1 * t4764) * t4794 + (t4686 * t4828 + t4723 * t4844) * t4795) * t4797;
  J_geo_dot(4,2) = -0.1e1 * t4949;
  J_geo_dot(2,2) = t4626 * t4791 + ((t4789 * t4816 + t5029) * t4790 + (-0.1e1 * t4998 - t5032) * t4796) * t4949;
  J_geo_dot(1,1) = (((t4662 + (t4997 - 0.1e1 * t4783) * t4788 + t4946) * t4795 + (-0.1e1 * t5003 - 0.1e1 * t5002) * t4792 + t4885 * t4788 + t4927 + t4830) * t4796 + (t4840 + t4913 - t5011) * t4795 + (-0.1e1 * t5020 - 0.1e1 * t5019 + t4750 - 0.1e1 * t4762) * t4794 + t4761 * t4987 + (-0.1e1 * t4772 * t4786 - 0.1e1 * t4760) * t4788 + t4762) * t4791 + (t4633 * t4795 + t5024) * t4797 + (((t4820 - t4842) * t4792 + t5041 * t4788 - t4786 * t4802 * t4863) * t4791 - t4797 * t4895) * t4790;
  J_geo_dot(5,3) = t4790 * t4949 + t4791 * t4954;
  J_geo_dot(6,1) = 0.0e0;
  J_geo_dot(3,3) = ((t4640 * t4794 + (-0.1e1 * t4695 * t4788 - 0.1e1 * t4769) * t4792 + (-t4787 * t4887 - 0.1e1 * t4694 * t4788) * t4786 + t4788 * t4888) * t4789 + (t4813 * t4966 + (t4788 * t4887 + t4942) * t4792 + (-0.1e1 * t4770 + t4938) * t4786 + 0.82500e-1 * t4801 - 0.1e1 * t4755) * t4795) * t4790 + (t5031 * t4789 + t4795 * t4816 + (t4821 - 0.384e0) * t4988) * t4954;
  J_geo_dot(5,7) = t4630 * t4791 + ((t4923 - 0.1e1 * t4990) * t4781 + t4795 * t4846 - 0.1e1 * t4870 + t4850 * t4793 + t4937 * t4789) * t4991 + ((t4734 + t4925) * t4794 + (t4845 + t4961) * t4795) * t4975;
  J_geo_dot(1,5) = -t5045 * t4838 + ((t4789 * t4962 + t4978) * t4793 + (t4797 * t4982 + (t4795 * t4962 - t4985) * t4794) * t4787) * t4915;
  J_geo_dot(6,2) = 0.0e0;
  J_geo_dot(1,4) = t4628 * t4797 + ((t4818 * t4792 + t5047 + t4854 - 0.1e1 * t4753) * t4788 + ((t4875 + t4999) * t4792 + (t4862 - 0.1e1 * t5009) * t4786 + t4831) * t4794 + (t4723 * t4794 * t4852 + t4686 * t4845) * t4795) * t4791;
  J_geo_dot(1,2) = t4626 * t4797 + ((-t4789 * t4851 - t4843 - t5029) * t4790 + (t4998 + t5032) * t4796) * t4951;
  J_geo_dot(1,6) = t4627 * t4797 + (-t4810 * t4916 + (-t4882 * t4907 + t4718) * t4978 + t4819 * t4979 + t4677 * t4974 - t4708 * t4985) * t4792 + (t4811 * t4916 + (t4710 + 0.88e-1 * t4846) * t4978 + t4818 * t4979 - t4682 * t4974 - t4721 * t4985) * t4786;
  J_geo_dot(6,6) = (t4815 * t4787 + (-0.1e1 * t4777 - 0.1e1 * t4801) * t4972) * t4790 + t4879 * t4787 * t4968 + t4735 * t4793 * t4796;
end

== matlab function Controller_damping_cbf_22Franka/Dynamic Parameters/Geometric Jacobian Derivative1 ==
  data: q_state input; J_geo_dot output; q_state_dot input
function J_geo_dot = Franka_J_geometric_dot(q_state, q_state_dot)
% Author: TU Wien, ACIN Robotics group
% Optimized and generated from Maple
  J_geo_dot = zeros(6,7);

  t213 = q_state_dot(2);
  t217 = q_state(4);
  t199 = sin(t217);
  t215 = q_state(6);
  t197 = sin(t215);
  t195 = 0.88e-1 * t197;
  t191 = t195 + 0.384e0;
  t203 = cos(t215);
  t300 = 0.1070e0 * t203;
  t446 = -t191 + t300;
  t455 = t446 * t199;
  t139 = -0.825e-1 - t455;
  t205 = cos(t217);
  t303 = 0.1070e0 * t197;
  t314 = 0.88e-1 * t203;
  t179 = t303 + t314;
  t216 = q_state(5);
  t204 = cos(t216);
  t251 = t179 * t204 - 0.825e-1;
  t428 = t251 * t205;
  t115 = -t428 + t139;
  t218 = q_state(3);
  t206 = cos(t218);
  t101 = t115 * t206;
  t198 = sin(t216);
  t200 = sin(t218);
  t416 = t200 * t198;
  t96 = t179 * t416 + t101;
  t466 = t96 * t213;
  t212 = q_state_dot(3);
  t465 = t115 * t212;
  t219 = q_state(2);
  t201 = sin(t219);
  t207 = cos(t219);
  t394 = t206 * t207;
  t108 = t201 * t446 - t251 * t394;
  t112 = t201 * t251 + t394 * t446;
  t214 = q_state_dot(1);
  t210 = q_state_dot(5);
  t421 = t179 * t198;
  t360 = t210 * t421;
  t209 = q_state_dot(6);
  t297 = 0.1070e0 * t209;
  t261 = t203 * t297;
  t310 = 0.88e-1 * t209;
  t268 = t197 * t310;
  t158 = t261 - t268;
  t425 = t158 * t204;
  t121 = t360 - t425;
  t211 = q_state_dot(4);
  t422 = t446 * t211;
  t157 = t179 * t209;
  t427 = t251 * t211;
  t452 = (t157 + t427) * t205;
  t225 = t452 - (t121 - t422) * t199;
  t423 = t446 * t205;
  t429 = t251 * t199;
  t246 = t423 - t429;
  t381 = t212 * t206;
  t464 = t246 * t381 + t214 * (t108 * t199 + t112 * t205) - t225 * t200;
  t463 = t96 * t214;
  t241 = t300 - 0.1e1 * t191;
  t264 = t197 * t297;
  t272 = t203 * t310;
  t378 = t213 * t206;
  t412 = t200 * t212;
  t461 = -t246 * t200 * t214 + (-0.1e1 * t112 * t199 + t108 * t205) * t211 + ((-0.1e1 * t446 * t378 - 0.1e1 * t360 + t425) * t205 + (t251 * t378 - t264 - t272) * t199) * t201 + ((-0.1e1 * t446 * t412 - 0.1e1 * t157 * t206) * t205 + (t121 * t206 + t251 * t412) * t199 + (t199 * t241 + t428) * t213) * t207;
  t326 = t198 * t381;
  t141 = t179 * t326;
  t402 = t204 * t210;
  t351 = t200 * t402;
  t459 = -t158 * t416 - t179 * t351 - t141 + 0.1e1 * t115 * t412;
  t382 = t211 * t205;
  t119 = t157 * t199 - t382 * t446;
  t417 = t199 * t211;
  t364 = t251 * t417;
  t447 = t119 + t364;
  t398 = t205 * t210;
  t249 = (t212 + t398) * t198;
  t401 = t204 * t211;
  t340 = t199 * t401;
  t453 = t249 + t340;
  t400 = t205 * t200;
  t342 = t204 * t400;
  t396 = t206 * t198;
  t162 = t342 + t396;
  t252 = -0.316e0 + t423;
  t231 = -0.1e1 * t429 + t252;
  t296 = 0.1070e0 * t210;
  t263 = t198 * t296;
  t309 = 0.88e-1 * t210;
  t274 = t198 * t309;
  t368 = t203 * t274 + t204 * t268;
  t117 = -t197 * t263 + t204 * t261 - t368;
  t432 = t117 * t205;
  t451 = t231 * t213 + (-t432 + t447) * t206;
  t289 = 0.10700e0 * t203;
  t163 = -t289 + t191;
  t450 = t163 * t199;
  t397 = t205 * t212;
  t294 = t210 + t397;
  t250 = t204 * t294;
  t220 = q_state(1);
  t202 = sin(t220);
  t387 = t207 * t214;
  t292 = t212 + t387;
  t448 = t292 * t202;
  t390 = t207 * t205;
  t333 = t206 * t390;
  t408 = t201 * t210;
  t357 = t199 * t408;
  t445 = t210 * t333 + t357;
  t444 = -t199 * t264 + t432;
  t339 = t205 * t381;
  t443 = t139 * t381 - 0.1e1 * t251 * t339;
  t442 = -0.1e1 * t428 + t139;
  t312 = 0.88e-1 * t205;
  t271 = t204 * t312;
  t302 = 0.1070e0 * t199;
  t166 = t271 + t302;
  t315 = 0.88e-1 * t200;
  t276 = t198 * t315;
  t131 = -t166 * t206 + t276;
  t299 = 0.1070e0 * t205;
  t313 = 0.88e-1 * t204;
  t167 = -t199 * t313 + t299;
  t100 = t131 * t207 + t167 * t201;
  t260 = t204 * t299;
  t298 = 0.1070e0 * t206;
  t124 = t198 * t298 - t199 * t315 + t200 * t260;
  t311 = 0.88e-1 * t206;
  t275 = t198 * t311;
  t301 = 0.1070e0 * t200;
  t125 = t199 * t301 + t200 * t271 + t275;
  t226 = t453 * t200;
  t237 = t206 * t250;
  t258 = t212 * t298;
  t295 = 0.1070e0 * t211;
  t259 = t205 * t295;
  t269 = t212 * t311;
  t308 = 0.88e-1 * t211;
  t270 = t205 * t308;
  t165 = -0.88e-1 * t199 + t260;
  t129 = -t165 * t206 + t198 * t301;
  t164 = t204 * t302 + t312;
  t99 = -t129 * t207 + t164 * t201;
  t441 = (t124 * t209 + t199 * t258 + t200 * t259 - t453 * t315 + 0.88e-1 * t237) * t197 + (t125 * t209 + t199 * t269 + t200 * t270 - t298 * t250 + 0.1070e0 * t226) * t203 - t214 * (t100 * t197 + t203 * t99);
  t169 = (0.13375e2 * t203 - 0.11e2 * t197) * t209;
  t440 = -0.8e-2 * t169;
  t439 = 0.8e-2 * t169;
  t190 = 0.13375e2 * t197 + 0.11e2 * t203;
  t438 = -0.8e-2 * t190;
  t437 = 0.8e-2 * t190;
  t436 = -0.4e-1 * t205;
  t189 = t199 * t272;
  t359 = t212 * t421;
  t265 = -t211 * t246 + t189 + t359 - t444;
  t138 = t158 * t396;
  t393 = t206 * t210;
  t336 = t204 * t393;
  t143 = t179 * t336;
  t373 = -t138 - t143;
  t433 = (t115 * t381 + t200 * t265 + t373) * t207;
  t262 = t199 * t295;
  t431 = (t204 * t262 + t205 * t263 + t270) * t206;
  t273 = t199 * t308;
  t430 = (-t204 * t273 - t205 * t274 + t259) * t206;
  t419 = t197 * t207;
  t418 = t199 * t210;
  t415 = t200 * t204;
  t414 = t200 * t207;
  t413 = t200 * t211;
  t410 = t201 * t199;
  t409 = t201 * t205;
  t407 = t201 * t214;
  t406 = t202 * t200;
  t405 = t203 * t199;
  t404 = t204 * t206;
  t403 = t204 * t209;
  t399 = t205 * t206;
  t395 = t206 * t199;
  t392 = t206 * t211;
  t391 = t207 * t199;
  t389 = t207 * t210;
  t388 = t207 * t212;
  t208 = cos(t220);
  t386 = t208 * t200;
  t384 = t209 * t197;
  t383 = t209 * t203;
  t380 = t213 * t200;
  t379 = t213 * t201;
  t377 = t213 * t207;
  t376 = t214 * t202;
  t375 = t214 * t208;
  t255 = t209 * t289;
  t290 = 0.10700e0 * t197;
  t256 = t210 * t290;
  t116 = t198 * t256 - t204 * t255 + t368;
  t140 = -t203 * t313 - t204 * t290 + 0.82500e-1;
  t374 = -t116 * t199 - t140 * t382;
  t358 = t199 * t413;
  t286 = t202 * t358;
  t337 = t206 * t375;
  t371 = t198 * t286 + t204 * t337;
  t243 = t309 * t415;
  t245 = t198 * t269;
  t370 = (t243 + t245) * t203;
  t181 = t203 * t276;
  t257 = t198 * t290;
  t369 = t200 * t257 + t181;
  t152 = t179 * t396;
  t94 = t115 * t200 - t152;
  t367 = t94 * t387;
  t366 = t94 * t379;
  t363 = t165 * t412;
  t362 = t166 * t412;
  t356 = t199 * t407;
  t355 = t202 * t400;
  t354 = t212 * t406;
  t353 = t214 * t400;
  t352 = t200 * t375;
  t350 = t201 * t376;
  t349 = t201 * t399;
  t348 = t211 * t410;
  t347 = t201 * t382;
  t346 = t201 * t412;
  t345 = t201 * t381;
  t344 = t203 * t382;
  t343 = t212 * t405;
  t341 = t204 * t399;
  t338 = t209 * t396;
  t335 = t204 * t414;
  t334 = t206 * t391;
  t332 = t208 * t377;
  t331 = t207 * t383;
  t330 = t207 * t382;
  t329 = t208 * t394;
  t328 = t205 * t384;
  t327 = t198 * t418;
  t325 = t199 * t379;
  t324 = t203 * t379;
  t323 = t208 * t379;
  t322 = t199 * t377;
  t321 = t200 * t377;
  t320 = t205 * t377;
  t319 = t206 * t377;
  t317 = t200 * t439;
  t170 = 0.2675e1 * t203 - 0.22e1 * t197 - 0.96e1;
  t316 = t170 * t436;
  t306 = -t140 * t199 + 0.316e0;
  t291 = t214 + t388;
  t288 = t140 * t205 - 0.82500e-1;
  t285 = t206 * t343;
  t284 = t200 * t344;
  t283 = t204 * t347;
  t282 = t204 * t322;
  t280 = t214 * t333;
  t279 = t199 * t200 * t384;
  t278 = t201 * t327;
  t277 = -0.1e1 * t392 + t213;
  t267 = -0.1e1 * t210 - 0.1e1 * t397;
  t266 = -0.1e1 * t212 - 0.1e1 * t398;
  t254 = t255 * t416 + t256 * t415 + t257 * t381 + t370;
  t253 = t204 * t212 * t386 + t376 * t404 + (t162 * t210 + t205 * t326) * t208;
  t248 = t291 * t206;
  t244 = t198 * t268;
  t240 = t267 * t206;
  t239 = t266 * t198;
  t238 = t266 * t206;
  t236 = t158 * t198 + t179 * t402;
  t161 = t333 + t410;
  t235 = (-0.1e1 * t378 + t211) * t198 * t205;
  t233 = -0.1e1 * t396 - 0.1e1 * t342;
  t228 = (t326 + t351) * t207;
  t230 = ((-0.1e1 * t363 - 0.1e1 * t431) * t207 + t129 * t379 + t100 * t209) * t203 + (-0.1e1 * t99 * t209 + (t362 - 0.1e1 * t430) * t207 - 0.1e1 * t131 * t379) * t197 + ((-0.1e1 * t326 - 0.1e1 * t351) * t207 - 0.1e1 * t278 + t282 + t283) * t300 + (t228 + t278 - 0.1e1 * t282 - 0.1e1 * t283) * t195 + t179 * (-0.1e1 * t348 + t320) + (-t124 * t203 + t125 * t197) * t214;
  t229 = t290 + t314;
  t224 = (-0.1e1 * t340 + t239) * t200;
  t223 = t199 * t277 + t200 * t267;
  t222 = ((t378 - 0.1e1 * t211) * t201 + t291 * t200) * t199;
  t221 = (-0.1e1 * t211 * t334 - 0.1e1 * t388 * t400 - 0.1e1 * t213 * t349 + t322 - 0.1e1 * t353 - 0.1e1 * t200 * t389 + t347) * t438 + t161 * t440;
  t160 = t416 - 0.1e1 * t341;
  t159 = -0.1e1 * t416 + t341;
  t156 = (-0.2675e1 * t197 - 0.22e1 * t203) * t209;
  t155 = t229 * t209;
  t127 = t161 * t198 + t335;
  t126 = t159 * t207 + t204 * t410;
  t113 = t163 * t205 + t306;
  t111 = t288 + t450;
  t110 = t316 + t306;
  t109 = -0.4e-1 * t170 * t199 + t288;
  t104 = t116 * t205;
  t98 = t126 * t197 + (t334 - 0.1e1 * t409) * t203;
  t97 = -0.82500e-1 + (-t229 * t204 + 0.82500e-1) * t205 + t450;
  t93 = t111 * t206 + t369;
  t92 = t109 * t206 + t369;
  t88 = t161 * t402 + (-0.1e1 * t204 * t380 + t235) * t201 + (t198 * t223 + t204 * t381) * t207;
  t84 = (-0.1e1 * t159 * t379 + (-0.1e1 * t357 + t207 * t238) * t198 + (t207 * t223 + t347) * t204) * t197 + t126 * t383 - 0.1e1 * t334 * t384 - 0.1e1 * t324 * t395 - 0.1e1 * t343 * t414 + t201 * t328 + (t206 * t330 - 0.1e1 * t320 + t348) * t203;
  J_geo_dot(1,5) = t371 * t438 + ((-0.1e1 * t200 * t323 - 0.1e1 * t210 * t355 - 0.1e1 * t376 * t414 + t212 * t329 - 0.1e1 * t354 + t445 * t208) * t438 + (t202 * t206 + t207 * t386) * t440) * t204 + (((-0.1e1 * t280 - 0.1e1 * t356 - 0.1e1 * t339 - 0.1e1 * t393) * t438 + t205 * t317) * t202 + t221 * t208) * t198;
  J_geo_dot(5,3) = t201 * t375 + t202 * t377;
  J_geo_dot(2,3) = ((-0.1e1 * t189 + t444) * t206 + t367 + (-0.1e1 * t429 + t241 * t205) * t392 + t459) * t208 + (0.1e1 * t463 + t433 - 0.1e1 * t366) * t202;
%   J_geo_dot(3,7) = 0.0e0;
  J_geo_dot(3,3) = -0.1e1 * t97 * t345 + (-0.1e1 * (0.384e0 * t382 + t189 - 0.82500e-1 * t417) * t201 - 0.1e1 * t97 * t377) * t200 + t203 * t275 * t377 + 0.88e-1 * ((-0.1e1 * t338 - 0.1e1 * (t211 + t403) * t400) * t197 + (t224 + t336) * t203) * t201 + (t338 - 0.1e1 * (-0.1e1 * t403 - 0.1e1 * t211) * t400) * t201 * t289 + (t198 * t319 + (t336 + ((-0.1e1 * t401 - 0.1e1 * t209) * t199 + t239) * t200) * t201) * t290;
  J_geo_dot(5,5) = ((-0.1e1 * t387 - 0.1e1 * t212) * t395 + (-0.1e1 * t413 + t407) * t205) * t208 + (t277 * t390 + t222) * t202;
  J_geo_dot(4,2) = -t375;
%   J_geo_dot(6,1) = 0.0e0;
  J_geo_dot(6,3) = -t379;
  J_geo_dot(2,4) = t202 * t461 + t208 * t464;
%   J_geo_dot(4,1) = 0.0e0;
  J_geo_dot(2,2) = (t110 * t207 + t201 * t92) * t375 + t202 * (((t104 + t211 * t316 + (-0.1e1 * t140 * t211 - 0.4e-1 * t156) * t199) * t206 - t109 * t412 - t200 * t244 + t254) * t201 + t92 * t377 + (t156 * t436 + 0.4e-1 * t170 * t417 + t374) * t207 - t110 * t379);
  J_geo_dot(1,3) = (-t366 + t433 + t463) * t208 + (-t367 + t265 * t206 + (t236 - t465) * t200) * t202;
  J_geo_dot(2,5) = t253 * t438 + ((t214 * t335 + (t280 - 0.1e1 * t358 + t356) * t198) * t438 + (t198 * t400 - 0.1e1 * t404) * t440) * t208 + (((-0.1e1 * t200 * t379 + t207 * t381 + t445) * t438 + t414 * t440) * t204 + t221 * t198) * t202;
  J_geo_dot(6,6) = (t235 + (t418 - 0.1e1 * t380) * t204) * t207 + (t204 * t238 + (t294 * t200 + (t392 - 0.1e1 * t213) * t199) * t198) * t201;
  J_geo_dot(1,2) = -(t113 * t207 + t201 * t93) * t376 + t208 * ((t93 * t213 - 0.1e1 * t163 * t417 + t155 * t205 + t374) * t207 + ((-0.1e1 * t140 * t417 + t163 * t382 + t155 * t199 + t104) * t206 - 0.1e1 * t113 * t213 + (-0.1e1 * t111 * t212 - t244) * t200 + t254) * t201);
%   J_geo_dot(1,7) = 0.0e0;
  J_geo_dot(6,7) = (t160 * t383 + (t197 * t250 + t343) * t200 + (-0.1e1 * t344 + ((t209 + t401) * t199 + t249) * t197) * t206) * t201 + (t160 * t197 - 0.1e1 * t203 * t395) * t377 - 0.1e1 * t327 * t419 + t207 * t328 + t205 * t324 + t203 * t211 * t391 + (t199 * t331 + (-0.1e1 * t325 + t330) * t197) * t204;
  J_geo_dot(3,2) = ((-t244 - 0.1e1 * t465) * t200 + t370 + t451) * t207 + (-0.1e1 * (t101 + t181) * t213 + (-0.1e1 * t157 - 0.1e1 * t427) * t205 + (-0.1e1 * t422 - 0.1e1 * t117) * t199) * t201 + t198 * t261 * t414 + (t228 - 0.1e1 * t379 * t416) * t303;
  J_geo_dot(5,2) = -0.1e1 * t376;
  J_geo_dot(5,7) = t84 * t202 + t98 * t375 + (-0.1e1 * t162 * t197 - 0.1e1 * t200 * t405) * t376 + ((t237 + t224) * t197 + t162 * t383 - 0.1e1 * t279 + t284 + t285) * t208;
  J_geo_dot(1,4) = -t202 * t464 + t208 * t461;
  J_geo_dot(6,5) = (-t213 + t392) * t409 + (-t346 + (-t211 + t378) * t207) * t199;
%   J_geo_dot(2,7) = 0.0e0;
  J_geo_dot(4,5) = t395 * t448 + t208 * t222 + ((-0.1e1 * t329 + t406) * t211 - 0.1e1 * t350 + t332) * t205;
  J_geo_dot(3,6) = ((-t131 * t209 + t198 * t258 + t296 * t415 + t363 + t431) * t203 + (-0.1e1 * t129 * t209 - 0.1e1 * t362 + t430 - 0.1e1 * t245 - 0.1e1 * t243) * t197) * t201 + (t129 * t203 - t131 * t197) * t377 + (-0.1e1 * t199 * t263 + t204 * t259 - 0.1e1 * t273) * t207 * t203 + (t199 * t274 - 0.1e1 * t204 * t270 - 0.1e1 * t262) * t419 + (-0.1e1 * t197 * t379 + t331) * t167 + (-0.1e1 * t324 - 0.1e1 * t207 * t384) * t164;
  J_geo_dot(1,1) = (t373 + t443) * t208 + t152 * t376 + ((t359 - 0.1e1 * t432 + t447) * t208 - 0.1e1 * t442 * t376) * t200 + (t96 * t375 + (-0.1e1 * t465 + t236) * t406 + (t141 + t451) * t202) * t207 + ((-0.1e1 * t466 - 0.1e1 * t157 * t205 - 0.1e1 * t446 * t417 - 0.1e1 * t117 * t199 - 0.1e1 * t251 * t382) * t202 + t231 * t375) * t201;
  J_geo_dot(2,1) = (((-0.1e1 * t364 + t432 - t119) * t206 + (-0.1e1 * t423 + t429 + 0.316e0) * t213 + t459) * t207 + (0.1e1 * t466 + t452 + (t117 + t422) * t199) * t201) * t208 - 0.1e1 * (-t207 * t96 + (-0.1e1 * t252 + t429) * t201) * t376 - 0.1e1 * t117 * t355 + t251 * t286 + t119 * t406 + (-0.1e1 * t337 + t354) * t421 + t442 * t352 + (-0.1e1 * t143 - 0.1e1 * t138 + t443) * t202;
  J_geo_dot(1,6) = t202 * t441 + t208 * t230;
  J_geo_dot(4,6) = (t88 - 0.1e1 * t198 * t353) * t208 + (-0.1e1 * t127 * t214 + t266 * t415 + t198 * t240) * t202 + t371;
  J_geo_dot(5,4) = t202 * t248 + (-0.1e1 * t202 * t379 + t292 * t208) * t200;
  J_geo_dot(4,4) = t208 * t248 + (-t323 - t448) * t200;
%   J_geo_dot(5,1) = 0.0e0;
  J_geo_dot(6,4) = -0.1e1 * t321 - 0.1e1 * t345;
%   J_geo_dot(3,1) = 0.0e0;
  J_geo_dot(2,6) = t202 * t230 - t208 * t441;
  J_geo_dot(3,5) = ((t210 * t349 - 0.1e1 * t199 * t389 + t321 + t345) * t437 + t201 * t317) * t204 + ((-0.1e1 * t206 * t348 + t325 - 0.1e1 * t200 * t408 - 0.1e1 * t330 + (-0.1e1 * t346 + t319) * t205) * t437 + (t349 - 0.1e1 * t391) * t439) * t198;
  J_geo_dot(4,3) = t332 - t350;
  J_geo_dot(5,6) = t127 * t375 + t88 * t202 + (-0.1e1 * t208 * t417 - 0.1e1 * t205 * t376) * t416 + t253;
  J_geo_dot(3,4) = (-t121 * t205 - t246 * t378 - t447) * t207 + (-(t455 + t428) * t213 + t225 * t206 + t246 * t412) * t201;
%   J_geo_dot(6,2) = 0.0e0;
  J_geo_dot(4,7) = t84 * t208 - 0.1e1 * t98 * t376 + t233 * t375 * t197 - 0.1e1 * t352 * t405 + ((t204 * t240 + t226) * t197 + t233 * t383 + t279 - 0.1e1 * t284 - 0.1e1 * t285) * t202;
end
